simulink model "stepperMotorADRCFirstOrderDataCollection"  (R2026a)
settings: Solver=FixedStepDiscrete  StopTime=0.06  FixedStep=5e-9
undefined symbols (not defined in the file): ADC_Offset, adc_volts_per_count, alpha_iqd, alpha_s, beta_iqd, beta_s, biq, bs, convert_adc_to_integer, electricalRadiansPerCount, gam_iqd, gam_s, k1_iqd, k1_s, KPth, loadcell_decode_gain, mechanicalRadiansPerCount, precise_step_radians, PWMVoltage, theta_ref
libraries: simulink x2, mcbeeMathTransformLib x2, hdlsllib x1
settings Model: DataTypeOverride=Off  Creator=mike  LastModifiedBy=drew
settings OptimizationCC: ConditionallyExecuteInputs=off
settings DebuggingCC: ParameterPrecisionLossMsg=none
settings HardwareCC: ProdHWDeviceType=ASIC/FPGA->ASIC/FPGA  TargetBitPerLong=64.0  TargetBitPerPointer=64.0  TargetBitPerSizeT=64.0  TargetBitPerPtrDiffT=64.0  TargetLongLongMode=on  TargetIntDivRoundTo=Zero  TargetEndianess=LittleEndian  TargetWordSize=64.0  TargetHWDeviceType=Custom Processor->MATLAB Host Computer  ProdEqTarget=off

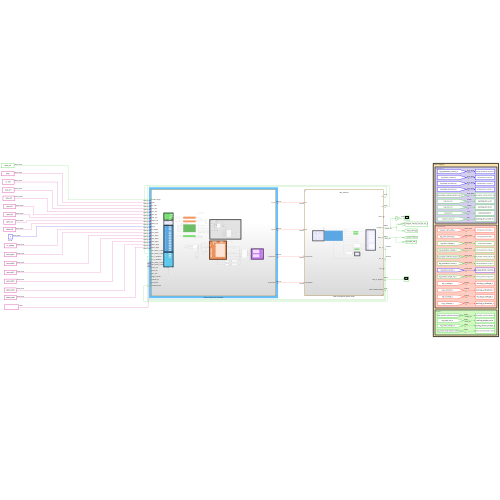
[thumbnail: Simulink's stored preview of the top-level diagram]
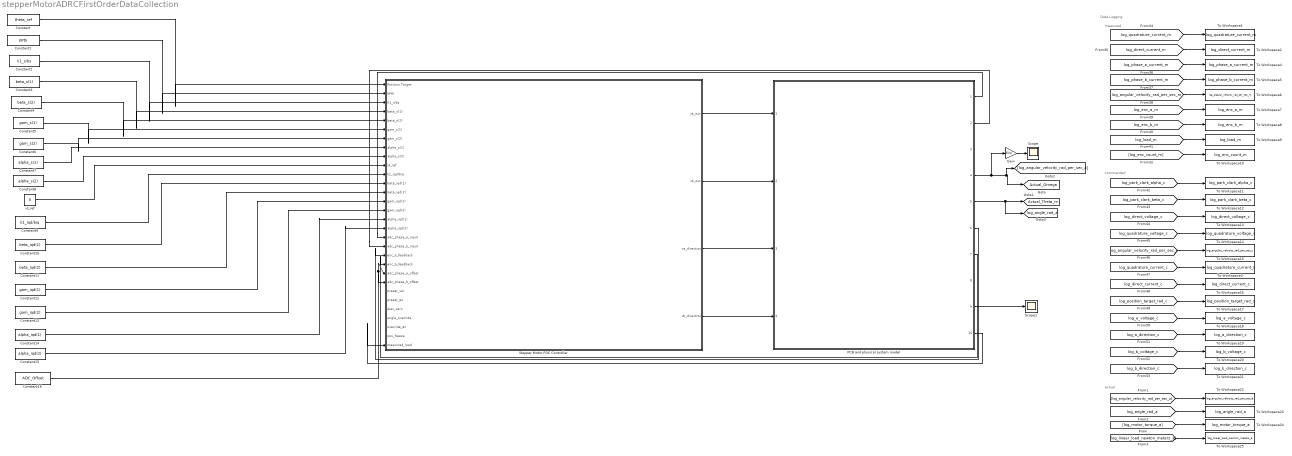
== system stepperMotorADRCFirstOrderDataCollection ==
  note: actual
  note: commanded
  note: measured
  note: Data Logging
  Constant : Constant  Value=theta_ref  OutDataTypeStr=PosType  SampleTime=-1
  Constant1 : Constant  Value=KPth  OutDataTypeStr=ParamType
  Constant10 : Constant  Value=beta_iqd(1)  OutDataTypeStr=ParamType
  Constant11 : Constant  Value=beta_iqd(2)  OutDataTypeStr=ParamType
  Constant12 : Constant  Value=gam_iqd(1)  OutDataTypeStr=ParamType
  Constant13 : Constant  Value=gam_iqd(2)  OutDataTypeStr=ParamType
  Constant14 : Constant  Value=alpha_iqd(1)  OutDataTypeStr=ParamType
  Constant15 : Constant  Value=alpha_iqd(2)  OutDataTypeStr=ParamType
  Constant16 : Constant  Value=ADC_Offset
  Constant2 : Constant  Value=k1_s/bs  OutDataTypeStr=ParamType
  Constant3 : Constant  Value=beta_s(1)  OutDataTypeStr=ParamType
  Constant4 : Constant  Value=beta_s(2)  OutDataTypeStr=ParamType
  Constant5 : Constant  Value=gam_s(1)  OutDataTypeStr=ParamType
  Constant6 : Constant  Value=gam_s(2)  OutDataTypeStr=ParamType
  Constant7 : Constant  Value=alpha_s(1)  OutDataTypeStr=ParamType
  Constant8 : Constant  Value=alpha_s(2)  OutDataTypeStr=ParamType
  Constant9 : Constant  Value=k1_iqd/biq  OutDataTypeStr=ParamType
  Gain : Gain  Gain=30/pi
  PCB and physical system model : Subsystem  ReferencedSubsystem=adrc_harness
  Scope : Scope
      settings: ActiveDisplayYMinimum=-42.844001916029548  ActiveDisplayYMaximum=385.596017244266  DataLoggingVariableName=ScopeData21
  Scope1 : Scope
      settings: Title=Actual Motor Position (Degrees)  ActiveDisplayYMinimum=117.68063353400193  ActiveDisplayYMaximum=118.08892845238269  YLabel=Degrees  DataLoggingVariableName=ScopeData8
  Stepper Motor FOC Controller : Subsystem
  To Workspace1 : ToWorkspace  VariableName=log_quadrature_current_m  SaveFormat=Timeseries  SampleTime=-1
  To Workspace10 : ToWorkspace  VariableName=log_enc_count_m  SaveFormat=Timeseries  SampleTime=-1
  To Workspace11 : ToWorkspace  VariableName=log_park_clark_alpha_c  SaveFormat=Timeseries  SampleTime=-1
  To Workspace12 : ToWorkspace  VariableName=log_park_clark_beta_c  SaveFormat=Timeseries  SampleTime=-1
  To Workspace13 : ToWorkspace  VariableName=log_direct_voltage_c  SaveFormat=Timeseries  SampleTime=-1
  To Workspace14 : ToWorkspace  VariableName=log_quadrature_voltage_c  SaveFormat=Timeseries  SampleTime=-1
  To Workspace15 : ToWorkspace  VariableName=log_angular_velocity_rad_per_sec_c  SaveFormat=Timeseries  SampleTime=-1
  To Workspace16 : ToWorkspace  VariableName=log_direct_current_c  SaveFormat=Timeseries  SampleTime=-1
  To Workspace17 : ToWorkspace  VariableName=log_position_target_rad_c  SaveFormat=Timeseries  SampleTime=-1
  To Workspace18 : ToWorkspace  VariableName=log_a_voltage_c  SaveFormat=Timeseries  SampleTime=-1
  To Workspace19 : ToWorkspace  VariableName=log_a_direction_c  SaveFormat=Timeseries  SampleTime=-1
  To Workspace2 : ToWorkspace  VariableName=log_direct_current_m  SaveFormat=Timeseries  SampleTime=-1
  To Workspace20 : ToWorkspace  VariableName=log_b_voltage_c  SaveFormat=Timeseries  SampleTime=-1
  To Workspace21 : ToWorkspace  VariableName=log_b_direction_c  SaveFormat=Timeseries  SampleTime=-1
  To Workspace22 : ToWorkspace  VariableName=log_angular_velocity_rad_per_sec_a  SaveFormat=Timeseries  SampleTime=-1
  To Workspace23 : ToWorkspace  VariableName=log_angle_rad_a  SaveFormat=Timeseries  SampleTime=-1
  To Workspace24 : ToWorkspace  VariableName=log_motor_torque_a  SaveFormat=Timeseries  SampleTime=-1
  To Workspace25 : ToWorkspace  VariableName=log_linear_load_newton_meters_a  SaveFormat=Timeseries  SampleTime=-1
  To Workspace3 : ToWorkspace  VariableName=log_quadrature_current_c  SaveFormat=Timeseries  SampleTime=-1
  To Workspace4 : ToWorkspace  VariableName=log_phase_a_current_m  SaveFormat=Timeseries  SampleTime=-1
  To Workspace5 : ToWorkspace  VariableName=log_phase_b_current_m  SaveFormat=Timeseries  SampleTime=-1
  To Workspace6 : ToWorkspace  VariableName=log_angular_velocity_rad_per_sec_m  SaveFormat=Timeseries  SampleTime=-1
  To Workspace7 : ToWorkspace  VariableName=log_enc_a_m  SaveFormat=Timeseries  SampleTime=-1
  To Workspace8 : ToWorkspace  VariableName=log_enc_b_m  SaveFormat=Timeseries  SampleTime=-1
  To Workspace9 : ToWorkspace  VariableName=log_load_m  SaveFormat=Timeseries  SampleTime=-1
  id_ref : Constant  Value=0  OutDataTypeStr=ParamType  SampleTime=-1
  tag scope: Actual_Omega=global, Actual_Theta_m=global, log_angle_rad_a=global
  wires:
  Constant/1 -> Stepper Motor FOC Controller/1(Position Target)
  Constant1/1 -> Stepper Motor FOC Controller/2(KPth)
  Constant2/1 -> Stepper Motor FOC Controller/3(K1_s/bs)
  Constant3/1 -> Stepper Motor FOC Controller/4(beta_s(1))
  Constant4/1 -> Stepper Motor FOC Controller/5(beta_s(2))
  Constant5/1 -> Stepper Motor FOC Controller/6(gam_s(1))
  Constant6/1 -> Stepper Motor FOC Controller/7(gam_s(2))
  Constant7/1 -> Stepper Motor FOC Controller/8(alpha_s(1))
  Constant8/1 -> Stepper Motor FOC Controller/9(alpha_s(2))
  id_ref/1 -> Stepper Motor FOC Controller/10(id_ref)
  Constant9/1 -> Stepper Motor FOC Controller/11(k1_iqd/biq)
  Constant10/1 -> Stepper Motor FOC Controller/12(beta_iqd(1))
  Constant11/1 -> Stepper Motor FOC Controller/13(beta_iqd(2))
  Constant12/1 -> Stepper Motor FOC Controller/14(gam_iqd(1))
  Constant13/1 -> Stepper Motor FOC Controller/15(gam_iqd(2))
  Constant14/1 -> Stepper Motor FOC Controller/16(alpha_iqd(1))
  Constant15/1 -> Stepper Motor FOC Controller/17(alpha_iqd(2))
  Stepper Motor FOC Controller/1(va_out) -> PCB and physical system model/1
  Stepper Motor FOC Controller/2(vb_out) -> PCB and physical system model/2
  PCB and physical system model/7 -> Stepper Motor FOC Controller/21(enc_b_feedback)
  PCB and physical system model/6 -> Stepper Motor FOC Controller/20(enc_a_feedback)
  PCB and physical system model/1 -> Stepper Motor FOC Controller/18(adc_phase_a_input)
  PCB and physical system model/2 -> Stepper Motor FOC Controller/19(adc_phase_b_input)
  PCB and physical system model/5 -> [log_angle_rad_a], [Actual_Theta_m]
  PCB and physical system model/9 -> Scope1/1
  Constant16/1 -> Stepper Motor FOC Controller/22(adc_phase_a_offset), Stepper Motor FOC Controller/23(adc_phase_b_offset)
  Stepper Motor FOC Controller/3(va_direction) -> PCB and physical system model/3
  Stepper Motor FOC Controller/4(vb_direction) -> PCB and physical system model/4
  PCB and physical system model/4 -> [log_angular_velocity_rad_per_sec_a], [Actual_Omega], Gain/1
  PCB and physical system model/10 -> Stepper Motor FOC Controller/30(measured_load)
  Gain/1 -> Scope/1
  [log_motor_torque_a] -> To Workspace24/1
  [log_direct_current_c] -> To Workspace16/1
  [log_a_direction_c] -> To Workspace19/1
  [log_quadrature_voltage_c] -> To Workspace14/1
  [log_park_clark_alpha_c] -> To Workspace11/1
  [log_quadrature_current_c] -> To Workspace3/1
  [log_b_direction_c] -> To Workspace21/1
  [log_a_voltage_c] -> To Workspace18/1
  [log_direct_voltage_c] -> To Workspace13/1
  [log_quadrature_current_m] -> To Workspace1/1
  [log_angular_velocity_rad_per_sec_c] -> To Workspace15/1
  [log_phase_a_current_m] -> To Workspace4/1
  [log_direct_current_m] -> To Workspace2/1
  [log_enc_count_m] -> To Workspace10/1
  [log_load_m] -> To Workspace9/1
  [log_enc_b_m] -> To Workspace8/1
  [log_position_target_rad_c] -> To Workspace17/1
  [log_enc_a_m] -> To Workspace7/1
  [log_park_clark_beta_c] -> To Workspace12/1
  [log_b_voltage_c] -> To Workspace20/1
  [log_phase_b_current_m] -> To Workspace5/1
  [log_angular_velocity_rad_per_sec_m] -> To Workspace6/1
  [log_angular_velocity_rad_per_sec_a] -> To Workspace22/1
  [log_angle_rad_a] -> To Workspace23/1
  [log_linear_load_newton_meters_a] -> To Workspace25/1

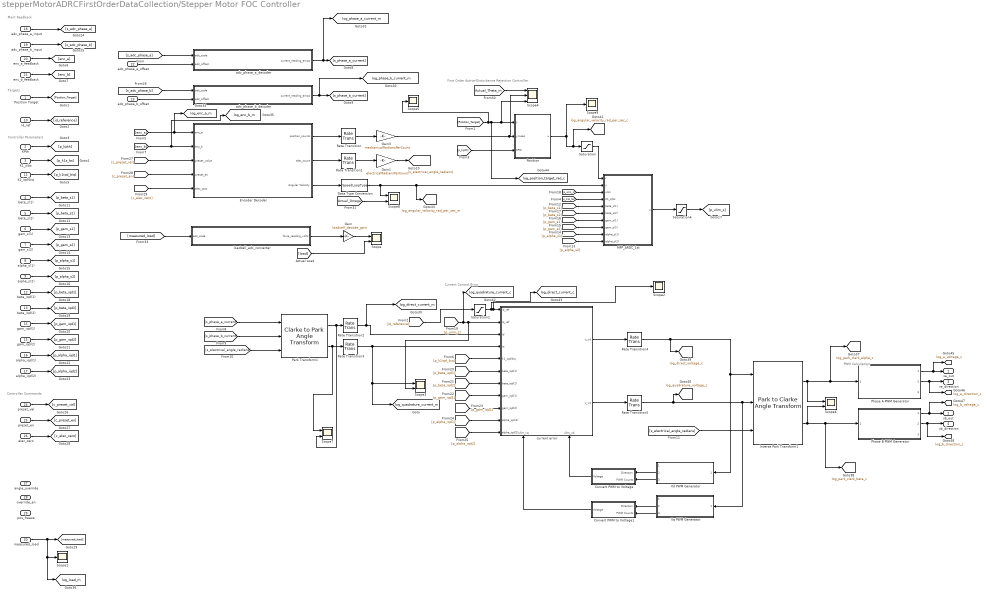
== system stepperMotorADRCFirstOrderDataCollection/Stepper Motor FOC Controller ==
  note: PWM Calculation
  note: Current Control Error
  note: Controller Commands
  note: Controller Parameters
  note: Targets
  note: Plant Feedback
  note: First Order Active-Disturbance Rejection Controller
  Position Target : Inport  OutDataTypeStr=PosType
  KPth : Inport  Port=2  OutDataTypeStr=ParamType
  K1_s/bs : Inport  Port=3  OutDataTypeStr=ParamType
  beta_s(1) : Inport  Port=4  OutDataTypeStr=ParamType
  beta_s(2) : Inport  Port=5  OutDataTypeStr=ParamType
  gam_s(1) : Inport  Port=6  OutDataTypeStr=ParamType
  gam_s(2) : Inport  Port=7  OutDataTypeStr=ParamType
  alpha_s(1) : Inport  Port=8  OutDataTypeStr=ParamType
  alpha_s(2) : Inport  Port=9  OutDataTypeStr=ParamType
  id_ref : Inport  Port=10  OutDataTypeStr=ParamType
  k1_iqd/biq : Inport  Port=11  OutDataTypeStr=ParamType
  beta_iqd(1) : Inport  Port=12  OutDataTypeStr=ParamType
  beta_iqd(2) : Inport  Port=13  OutDataTypeStr=ParamType
  gam_iqd(1) : Inport  Port=14  OutDataTypeStr=ParamType
  gam_iqd(2) : Inport  Port=15  OutDataTypeStr=ParamType
  alpha_iqd(1) : Inport  Port=16  OutDataTypeStr=ParamType
  alpha_iqd(2) : Inport  Port=17  OutDataTypeStr=ParamType
  adc_phase_a_input : Inport  Port=18
  adc_phase_b_input : Inport  Port=19
  enc_a_feedback : Inport  Port=20
  enc_b_feedback : Inport  Port=21
  adc_phase_a_offset : Inport  Port=22  OutDataTypeStr=uint16
  adc_phase_b_offset : Inport  Port=23  OutDataTypeStr=uint16
  preset_val : Inport  Port=24  OutDataTypeStr=fixdt(1,32,0)
  preset_en : Inport  Port=25  OutDataTypeStr=boolean
  elec_zero : Inport  Port=26  OutDataTypeStr=boolean
  angle_override : Inport  Port=27  OutDataTypeStr=uint16
  override_en : Inport  Port=28  OutDataTypeStr=boolean
  pos_freeze : Inport  Port=29  OutDataTypeStr=boolean
  measured_load : Inport  Port=30
  Convert PWM to Voltage : Subsystem
  Convert PWM to Voltage1 : Subsystem
  Data Type Conversion : DataTypeConversion  OutDataTypeStr=SpeedLoopType  SaturateOnIntegerOverflow=off  RndMeth=Floor
  Encoder Decoder : Subsystem
  Gain : Gain  Gain=loadcell_decode_gain  OutDataTypeStr=ParamType
  Gain1 : Gain  Gain=electricalRadiansPerCount  OutDataTypeStr=PosType  SaturateOnIntegerOverflow=on
  Gain3 : Gain  Gain=mechanicalRadiansPerCount  OutDataTypeStr=PosType  SaturateOnIntegerOverflow=on
  Inverse Park Transform1 : mcbeeMathTransformLib/Park to Clarke Angle Transform  AxisAlignment=D-axis  UseWithEmbedded=on  PhaseInput=Two inputs  ThetaInput=Electrical position  AngleInput=Radians  N_points=1024
      settings: LibrarySourceBlock=mcbhdllib/Controls/Math Transforms/Inverse Park Transform
  MFP_ARDC_1st : Subsystem
  Park Transform1 : mcbeeMathTransformLib/Clarke to Park Angle Transform  AxisAlignment=D-axis  UseWithEmbedded=on  PhaseInput=Two inputs  ThetaInput=Electrical position  AngleInput=Radians  N_points=1024
      settings: LibrarySourceBlock=mcbhdllib/Controls/Math Transforms/Park Transform
  Phase A PWM Generator : Subsystem  ReferencedSubsystem=PWM_Generator
  Phase B PWM Generator : Subsystem  ReferencedSubsystem=PWM_Generator
  "Position " : Subsystem
  Rate Transition{,1..3} (4 alike) : RateTransition  OutPortSampleTime=2e-5
  Rate Transition4 : RateTransition  OutPortSampleTime=1e-7
  Rate Transition5 : RateTransition  OutPortSampleTime=1e-7
  Saturation : Saturate  UpperLimit=35.5  LowerLimit=-35.5
  Saturation2 : Saturate  UpperLimit=2.4  LowerLimit=-2.4  OutDataTypeStr=ParamType
  Saturation4 : Saturate  UpperLimit=4.16  LowerLimit=-4.16
  Scope{,3,6..8} (5 alike) : Scope  NumInputPorts=2
      Scope settings: Title=Calculated Load and Torque Load  ActiveDisplayYMinimum=-0.011365323760298198  ActiveDisplayYMaximum=0.10228791384268379
      Scope3 settings: Title=Measured Iq vs Iq Reference  ActiveDisplayYMinimum=-7.8918533325195312  ActiveDisplayYMaximum=11.987983703613281  YLabel=Amps  DataLoggingVariableName=ScopeData20
      Scope6 settings: Title="Output  Voltages"  ActiveDisplayYMinimum=-1  ActiveDisplayYMaximum=1  DataLoggingVariableName=ScopeData9  DataLoggingSaveFormat=Array
      Scope7 settings: ActiveDisplayYMinimum=-1  ActiveDisplayYMaximum=1  DataLoggingVariableName=ScopeData26
      Scope8 settings: Title=Calculated and Actual Velocity  ActiveDisplayYMinimum=5.2986835943204227  ActiveDisplayYMaximum=29.84236950740636  YLabel=Radians/Second  DataLoggingVariableName=ScopeData23  DataLoggingSaveFormat=Array
  Scope{1..2,5,9} (4 alike) : Scope
      Scope1 settings: ActiveDisplayYMinimum=-1  ActiveDisplayYMaximum=1  DataLoggingVariableName=ScopeData5
      Scope2 settings: ActiveDisplayYMinimum=-1  ActiveDisplayYMaximum=1  DataLoggingVariableName=ScopeData22
      Scope5 settings: ActiveDisplayYMinimum=-1  ActiveDisplayYMaximum=1  DataLoggingVariableName=ScopeData25
      Scope9 settings: Title=Output of Position Controller  ActiveDisplayYMinimum=21899.960541585759  ActiveDisplayYMaximum=43949.960541585751  YLabel=Radians  DataLoggingVariableName=ScopeData24  DataLoggingSaveFormat=Array
  Scope4 : Scope  NumInputPorts=3
      settings: Title=Position Debugging  ActiveDisplayYMinimum=-0.035609373496401926  ActiveDisplayYMaximum=0.32048436146761738  YLabel=Radians  DataLoggingVariableName=ScopeData7  DataLoggingSaveFormat=Array
  Vd PWM Generator : Subsystem  ReferencedSubsystem=PWM_Generator
  Vq PWM Generator : Subsystem  ReferencedSubsystem=PWM_Generator
  adc_phase_a_decoder : Subsystem
  adc_phase_b_decoder : Subsystem
  current error : Subsystem
      settings: PortSchema="{\"entries\":[{\"content\":{\"sides\":[{\"content\":{\"connectorIds\":[\"In1\",\"In2\",\"In3\",\"In4\",\"In5\",\"In6\",\"In7\",\"In8\",\"In9\",\"In10\",\"In11\"]},\"type\":\"ConnectorPlacement.EquallySpacedRectSide\",\"uuid\":\"1b67f1ba-d970-4a72-948b-8a645885f311\"},{\"content\":{\"connectorIds\":[\"Out1\",\"Out2\"],\"side\":\"RIGHT\"},\"type\":\"ConnectorPlacement.EquallySpacedRectSide\",\"uuid\":\"43bd9de9-c038-41d9-a38f-2b3bf68f84b7\"},{\"content\":{\"side\":\"TOP\"},\"type\":\"ConnectorPlacement.EquallySpacedRectSide\",\"uuid\":\"199b5c60-7e13-4435-9b33-d3faaa781c81\"},{\"content\":{\"connectorIds\":[\"In12\",\"In13\"],\"side\":\"BOTTOM\"},\"type\":\"ConnectorPlacement.EquallySpacedRectSide\",\"uuid\":\"8463aca4-e427-4dc0-a0b4-e373bcd68b49\"}]},\"type\":\"ConnectorPlacement.EquallySpacedConnector\",\"uuid\":\"7665834e-14df-482a-91d4-36c3c32286ac\"}],\"packageUris\":[\"http://schema.mathworks.com/mf0/Connector/R2020b\"],\"version\":\"1.0\"}"
  loadcell_adc_converter : Subsystem
  va_out : Outport  OutDataTypeStr=boolean
  vb_out : Outport  Port=2  OutDataTypeStr=boolean
  va_direction : Outport  Port=3  OutDataTypeStr=boolean
  vb_direction : Outport  Port=4  OutDataTypeStr=boolean
  tag scope: log_a_direction_c=global, log_a_voltage_c=global, log_angular_velocity_rad_per_sec_c=global, log_angular_velocity_rad_per_sec_m=global, log_b_direction_c=global, log_b_voltage_c=global, log_direct_current_c=global, log_direct_current_m=global, log_direct_voltage_c=global, log_enc_a_m=global, log_enc_b_m=global, log_load_m=global, log_park_clark_alpha_c=global, log_park_clark_beta_c=global, log_phase_a_current_m=global, log_phase_b_current_m=global, log_position_target_rad_c=global, log_quadrature_current_c=global, log_quadrature_current_m=global, log_quadrature_voltage_c=global
  wires:
  [Position_Target] -> Scope5/1, [log_position_target_rad_c], Scope4/3, "Position "/1(y)
  Inverse Park Transform1/1 -> [log_park_clark_alpha_c], Phase A PWM Generator/1, Scope6/1
  Position Target/1 -> [Position_Target]
  id_ref/1 -> [id_reference]
  [p_kpth] -> "Position "/3(KPth)
  KPth/1 -> [p_kpth]
  [p_k1s_bs] -> MFP_ARDC_1st/4(K1_s/bs)
  K1_s/bs/1 -> [p_k1s_bs]
  [p_k1iqd_biq] -> current error/5(k1_iqd/biq)
  k1_iqd/biq/1 -> [p_k1iqd_biq]
  adc_phase_a_offset/1 -> adc_phase_a_decoder/2(adc_offset)
  adc_phase_b_offset/1 -> adc_phase_b_decoder/2(adc_offset)
  enc_a_feedback/1 -> [enc_a]
  enc_b_feedback/1 -> [enc_b]
  [enc_a] -> [log_enc_a_m], Encoder Decoder/1(enc_a)
  [enc_b] -> [log_enc_b_m], Encoder Decoder/2(enc_b)
  adc_phase_a_decoder/1(current_reading_amps) -> [log_phase_a_current_m], [s_phase_a_current]
  adc_phase_b_decoder/1(current_reading_amps) -> [log_phase_b_current_m], [s_phase_b_current]
  [s_phase_a_current] -> Park Transform1/1
  [s_phase_b_current] -> Park Transform1/2
  [s_electrical_angle_radians] -> Park Transform1/3
  [s_electrical_angle_radians] -> Inverse Park Transform1/3
  [p_beta_s1] -> MFP_ARDC_1st/5(beta_s(1))
  [p_beta_s2] -> MFP_ARDC_1st/6(beta_s(2))
  [p_gam_s1] -> MFP_ARDC_1st/7(gam_s(1))
  [p_gam_s2] -> MFP_ARDC_1st/8(gam_s(2))
  [p_alpha_s1] -> MFP_ARDC_1st/9(alpha_s(1))
  [p_alpha_s2] -> MFP_ARDC_1st/10(alpha_s(2))
  alpha_s(2)/1 -> [p_alpha_s2]
  alpha_s(1)/1 -> [p_alpha_s1]
  gam_s(2)/1 -> [p_gam_s2]
  gam_s(1)/1 -> [p_gam_s1]
  beta_s(2)/1 -> [p_beta_s2]
  beta_s(1)/1 -> [p_beta_s1]
  MFP_ARDC_1st/1(u) -> Saturation4/1
  [p_ulim_s] -> MFP_ARDC_1st/3(ulim)
  beta_iqd(1)/1 -> [p_beta_iqd1]
  beta_iqd(2)/1 -> [p_beta_iqd2]
  [p_beta_iqd2] -> current error/7(beta_iqd(2))
  [p_beta_iqd1] -> current error/6(beta_iqd(1))
  gam_iqd(2)/1 -> [p_gam_iqd2]
  gam_iqd(1)/1 -> [p_gam_iqd1]
  [p_gam_iqd1] -> current error/8(gam_iqd(1))
  [p_gam_iqd2] -> current error/9(gam_iqd(2))
  [p_alpha_iqd1] -> current error/10(alpha_iqd(1))
  [p_alpha_iqd2] -> current error/11(alpha_iqd(2))
  alpha_iqd(1)/1 -> [p_alpha_iqd1]
  alpha_iqd(2)/1 -> [p_alpha_iqd2]
  adc_phase_a_input/1 -> [s_adc_phase_a]
  adc_phase_b_input/1 -> [s_adc_phase_b]
  [s_adc_phase_a] -> adc_phase_a_decoder/1(adc_code)
  [s_adc_phase_b] -> adc_phase_b_decoder/1(adc_code)
  [c_elec_zero] -> Encoder Decoder/5(elec_zero)
  [c_preset_en] -> Encoder Decoder/4(preset_en)
  [c_preset_val] -> Encoder Decoder/3(preset_value)
  elec_zero/1 -> [c_elec_zero]
  preset_en/1 -> [c_preset_en]
  preset_val/1 -> [c_preset_val]
  Saturation2/1 -> Scope2/1, [log_direct_current_c], current error/1(id_ref)
  Rate Transition/1 -> Gain3/1
  Rate Transition1/1 -> Gain1/1
  Gain1/1 -> [s_electrical_angle_radians]
  Gain3/1 -> "Position "/2(ymeas), Scope4/2
  current error/1(u_vd) -> Rate Transition4/1
  Saturation4/1 -> [p_ulim_s]
  Park Transform1/1 -> Scope7/2, Rate Transition2/1
  Park Transform1/2 -> Scope7/1, Rate Transition3/1
  current error/2(u_vq) -> Rate Transition5/1
  Encoder Decoder/1(position_counts) -> Rate Transition/1
  Encoder Decoder/2(elec_count) -> Rate Transition1/1
  "Position "/1(u) -> [log_angular_velocity_rad_per_sec_c], Saturation/1, Scope9/1
  Encoder Decoder/3(Angular Velocity) -> Data Type Conversion/1
  Phase A PWM Generator/1 -> [log_a_voltage_c], va_out/1
  Phase A PWM Generator/2 -> [log_a_direction_c], va_direction/1
  Phase B PWM Generator/2 -> [log_b_direction_c], vb_direction/1
  Phase B PWM Generator/1 -> [log_b_voltage_c], vb_out/1
  Convert PWM to Voltage1/1(Voltage) -> current error/12(ulim_vq)
  Rate Transition4/1 -> [log_direct_voltage_c], Vd PWM Generator/1, Inverse Park Transform1/1
  Rate Transition5/1 -> [log_quadrature_voltage_c], Inverse Park Transform1/2, Vq PWM Generator/1
  [p_ulim_s] -> [log_quadrature_current_c], Scope3/2, current error/2(iq_ref)
  Data Type Conversion/1 -> [log_angular_velocity_rad_per_sec_m], MFP_ARDC_1st/2(y), Scope8/1
  Inverse Park Transform1/2 -> Scope6/2, [log_park_clark_beta_c], Phase B PWM Generator/1
  [Actual_Theta_m] -> Scope4/1
  Convert PWM to Voltage/1(Voltage) -> current error/13(ulim_vd)
  Vd PWM Generator/2 -> Convert PWM to Voltage/1(Direction)
  Vd PWM Generator/3 -> Convert PWM to Voltage/2(PWM Counts)
  Vq PWM Generator/3 -> Convert PWM to Voltage1/2(PWM Counts)
  Vq PWM Generator/2 -> Convert PWM to Voltage1/1(Direction)
  measured_load/1 -> [log_load_m], Scope1/1, [measured_load]
  loadcell_adc_converter/1(force_reading_volts) -> Gain/1
  [load] -> Scope/2
  [measured_load] -> loadcell_adc_converter/1(adc_code)
  Saturation/1 -> MFP_ARDC_1st/1(r)
  [Actual_Omega] -> Scope8/2
  Rate Transition3/1 -> [log_quadrature_current_m], Scope3/1, current error/4(iq)
  Rate Transition2/1 -> [log_direct_current_m], current error/3(id)
  [id_reference] -> Saturation2/1
  Gain/1 -> Scope/1

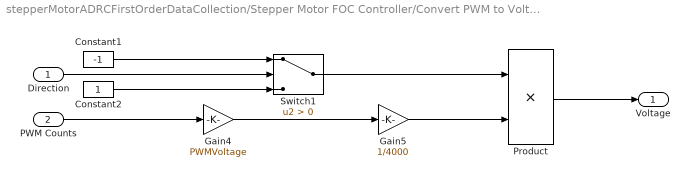
== system stepperMotorADRCFirstOrderDataCollection/Stepper Motor FOC Controller/Convert PWM to Voltage ==
  Direction : Inport
  PWM Counts : Inport  Port=2
  Constant1 : Constant  Value=-1
  Constant2 : Constant
  Gain4 : Gain  Gain=PWMVoltage
  Gain5 : Gain  Gain=1/4000
  Product : Product
  Switch1 : Switch  Criteria=u2 > Threshold  SaturateOnIntegerOverflow=off  InputSameDT=off
  Voltage : Outport
  wires:
  Gain4/1 -> Gain5/1
  Gain5/1 -> Product/2
  Switch1/1 -> Product/1
  Constant1/1 -> Switch1/1
  Constant2/1 -> Switch1/3
  PWM Counts/1 -> Gain4/1
  Direction/1 -> Switch1/2
  Product/1 -> Voltage/1

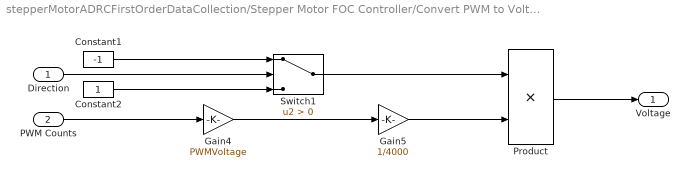
== system stepperMotorADRCFirstOrderDataCollection/Stepper Motor FOC Controller/Convert PWM to Voltage1 ==
  Direction : Inport
  PWM Counts : Inport  Port=2
  Constant1 : Constant  Value=-1
  Constant2 : Constant
  Gain4 : Gain  Gain=PWMVoltage
  Gain5 : Gain  Gain=1/4000
  Product : Product
  Switch1 : Switch  Criteria=u2 > Threshold  SaturateOnIntegerOverflow=off  InputSameDT=off
  Voltage : Outport
  wires:
  Gain4/1 -> Gain5/1
  Gain5/1 -> Product/2
  Switch1/1 -> Product/1
  Constant1/1 -> Switch1/1
  Constant2/1 -> Switch1/3
  PWM Counts/1 -> Gain4/1
  Direction/1 -> Switch1/2
  Product/1 -> Voltage/1

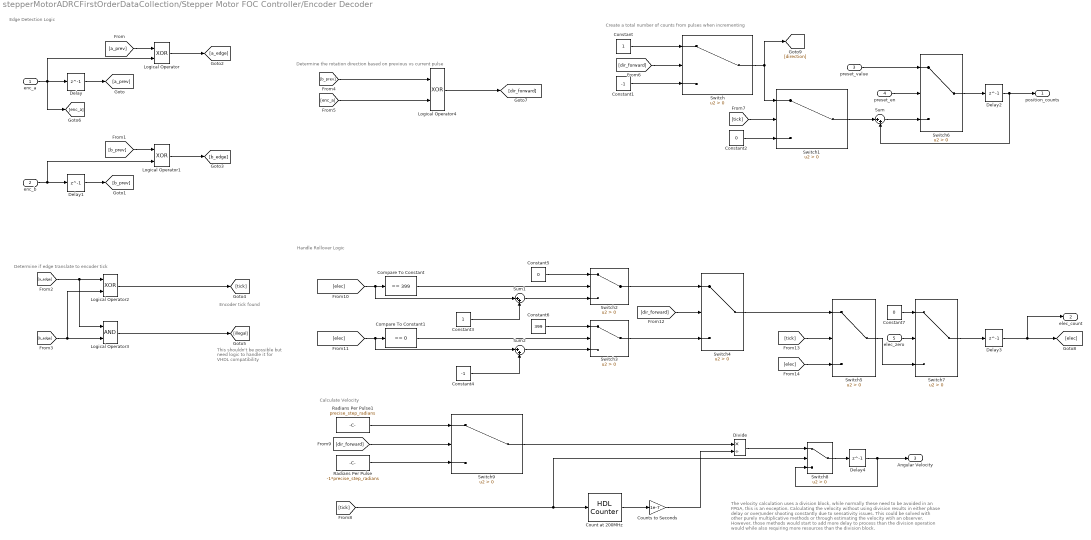
== system stepperMotorADRCFirstOrderDataCollection/Stepper Motor FOC Controller/Encoder Decoder ==
  note: The velocity calculation uses a division block, while normally these need to be avoided in an FPGA, this is an exception. Calculating the velocity without using division results in either phase delay or over/under shooting constantly due to sensativity issues. This could be solved with other purely multiplicative methods or through estimating the velocity wtih an observer. However, those methods would start to add more delay to process than the division operation would while also requiring more resources than the division block.
  note: Calculate Velocity
  note: Handle Rollover Logic
  note: Create a total number of counts from pulses when incrementing
  note: Determine the rotation direction based on previous vs current pulse
  note: Encoder tick found
  note: Determine if edge translate to encoder tick
  note: Edge Detection Logic
  note: This shouldn't be possible but need logic to handle it for VHDL compatibility
  enc_a : Inport  OutDataTypeStr=boolean
  enc_b : Inport  Port=2  OutDataTypeStr=boolean
  preset_value : Inport  Port=3  OutDataTypeStr=fixdt(1,32,0)
  preset_en : Inport  Port=4  OutDataTypeStr=boolean
  elec_zero : Inport  Port=5  OutDataTypeStr=boolean
  Compare To Constant : simulink/Logic and Bit Operations/Compare To Constant  relop===  const=399  OutDataTypeStr=boolean
  Compare To Constant1 : simulink/Logic and Bit Operations/Compare To Constant  relop===  const=0  OutDataTypeStr=boolean
  Constant : Constant  OutDataTypeStr=int32
  Constant1 : Constant  Value=-1  OutDataTypeStr=int32
  Constant2 : Constant  Value=0  OutDataTypeStr=int32
  Constant3 : Constant  OutDataTypeStr=int32
  Constant4 : Constant  Value=-1  OutDataTypeStr=int32
  Constant5 : Constant  Value=0  OutDataTypeStr=int32
  Constant6 : Constant  Value=399  OutDataTypeStr=int32
  Constant7 : Constant  Value=0  OutDataTypeStr=int32
  Count at 200MHz : hdlsllib/Sources/HDL Counter  CountType=Count limited  CountInit=0  CountStep=1  CountMax=199999999  CountFromType=Initial value  CountFrom=0  CountResetPort=on  CountLoadPort=off  CountEnbPort=off  CountDirPort=off  CountHitOutputPort=off  CountDataType=Unsigned  CountWordLen=32  CountFracLen=0  CountSampTime=5e-9
  Counts to Seconds : Gain  Gain=1e-7  OutDataTypeStr=VelType
  Delay{,1..4} (5 alike) : Delay  DelayLength=1  InputProcessing=Columns as channels (frame based)  SampleTime=1e-7
  Divide : Product  Inputs=*/  OutDataTypeStr=VelType  SaturateOnIntegerOverflow=on
  Logical Operator{,1..2,4} (4 alike) : Logic  Operator=XOR  AllPortsSameDT=off  OutDataTypeStr=boolean
  Logical Operator3 : Logic  AllPortsSameDT=off  OutDataTypeStr=boolean
  Radians Per Pulse : Constant  Value=-1*precise_step_radians  OutDataTypeStr=VelType
  Radians Per Pulse1 : Constant  Value=precise_step_radians  OutDataTypeStr=VelType
  Sum : Sum  Inputs=|++  OutDataTypeStr=int32  SaturateOnIntegerOverflow=on
  Sum1 : Sum  Inputs=|++  OutDataTypeStr=int32
  Sum2 : Sum  Inputs=|++  OutDataTypeStr=int32
  Switch{,1..5} (6 alike) : Switch  Criteria=u2 > Threshold  SaturateOnIntegerOverflow=off  InputSameDT=off
  Switch6 : Switch  Criteria=u2 > Threshold  OutDataTypeStr=CountType  SaturateOnIntegerOverflow=off  InputSameDT=off
  Switch7 : Switch  Criteria=u2 > Threshold  OutDataTypeStr=CountType  SaturateOnIntegerOverflow=off  InputSameDT=off
  Switch8 : Switch  Criteria=u2 > Threshold  OutDataTypeStr=VelType  SaturateOnIntegerOverflow=off  InputSameDT=off
  Switch9 : Switch  Criteria=u2 > Threshold  OutDataTypeStr=VelType  SaturateOnIntegerOverflow=off  InputSameDT=off
  position_counts : Outport  OutDataTypeStr=CountType
  elec_count : Outport  Port=2  OutDataTypeStr=CountType
  Angular Velocity : Outport  Port=3  OutDataTypeStr=VelType
  wires:
  enc_b/1 -> Logical Operator1/2, Delay1/1
  enc_a/1 -> [enc_a], Logical Operator/2, Delay/1
  Delay/1 -> [a_prev]
  Delay1/1 -> [b_prev]
  [b_prev] -> Logical Operator1/1
  [a_prev] -> Logical Operator/1
  Logical Operator/1 -> [a_edge]
  Logical Operator1/1 -> [b_edge]
  [b_edge] -> Logical Operator3/2, Logical Operator2/2
  [a_edge] -> Logical Operator2/1, Logical Operator3/1
  Logical Operator2/1 -> [tick]
  Logical Operator3/1 -> [illegal]
  [b_prev] -> Logical Operator4/1
  [enc_a] -> Logical Operator4/2
  Logical Operator4/1 -> [dir_forward]
  Constant/1 -> Switch/1
  Constant1/1 -> Switch/3
  [dir_forward] -> Switch/2
  [tick] -> Switch1/2
  Constant2/1 -> Switch1/3
  Switch/1 -> Switch1/1, [direction]
  Switch1/1 -> Sum/1
  Delay2/1 -> position_counts/1, Sum/2
  Constant5/1 -> Switch2/1
  Compare To Constant1/1 -> Switch3/2
  Sum2/1 -> Switch3/3
  Sum1/1 -> Switch2/3
  Constant6/1 -> Switch3/1
  [elec] -> Sum2/1, Compare To Constant1/1
  [elec] -> Sum1/1, Compare To Constant/1
  Switch2/1 -> Switch4/1
  Constant3/1 -> Sum1/2
  Compare To Constant/1 -> Switch2/2
  Constant4/1 -> Sum2/2
  [dir_forward] -> Switch4/2
  Switch3/1 -> Switch4/3
  Switch4/1 -> Switch5/1
  [tick] -> Switch5/2
  [elec] -> Switch5/3
  Delay3/1 -> elec_count/1, [elec]
  Sum/1 -> Switch6/3
  Switch6/1 -> Delay2/1
  preset_en/1 -> Switch6/2
  preset_value/1 -> Switch6/1
  Constant7/1 -> Switch7/1
  elec_zero/1 -> Switch7/2
  Switch5/1 -> Switch7/3
  Switch7/1 -> Delay3/1
  Count at 200MHz/1 -> Counts to Seconds/1
  Switch8/1 -> Delay4/1
  Delay4/1 -> Angular Velocity/1, Switch8/3
  Counts to Seconds/1 -> Divide/2
  Switch9/1 -> Divide/1
  Radians Per Pulse/1 -> Switch9/3
  Radians Per Pulse1/1 -> Switch9/1
  Divide/1 -> Switch8/1
  [dir_forward] -> Switch9/2
  [tick] -> Switch8/2, Count at 200MHz/1

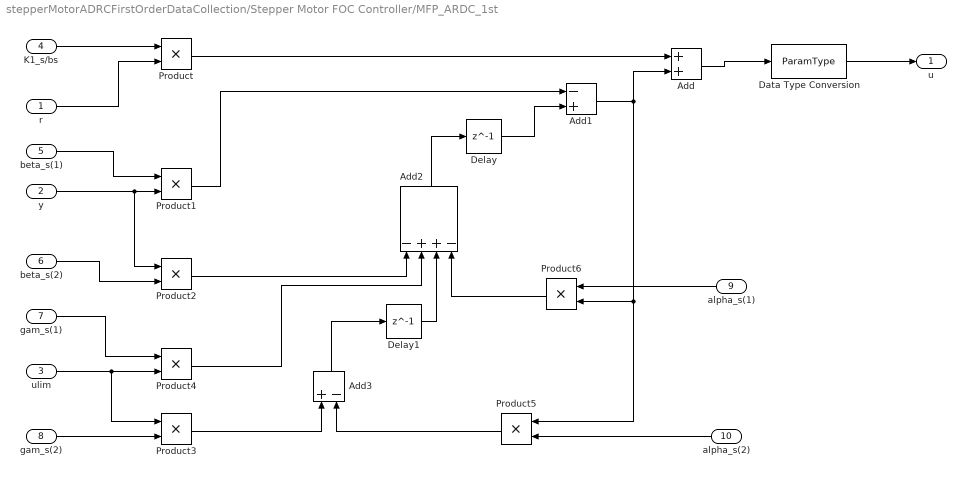
== system stepperMotorADRCFirstOrderDataCollection/Stepper Motor FOC Controller/MFP_ARDC_1st ==
  r : Inport  OutDataTypeStr=PosType
  y : Inport  Port=2  OutDataTypeStr=PosType
  ulim : Inport  Port=3  OutDataTypeStr=ParamType
  K1_s/bs : Inport  Port=4  OutDataTypeStr=ParamType
  beta_s(1) : Inport  Port=5  OutDataTypeStr=ParamType
  beta_s(2) : Inport  Port=6  OutDataTypeStr=ParamType
  gam_s(1) : Inport  Port=7  OutDataTypeStr=ParamType
  gam_s(2) : Inport  Port=8  OutDataTypeStr=ParamType
  alpha_s(1) : Inport  Port=9  OutDataTypeStr=ParamType
  alpha_s(2) : Inport  Port=10  OutDataTypeStr=ParamType
  Add : Sum  OutDataTypeStr=SpeedLoopType  SaturateOnIntegerOverflow=on
  Add1 : Sum  Inputs=-+  OutDataTypeStr=SpeedLoopType  SaturateOnIntegerOverflow=on
  Add2 : Sum  Inputs=-++-  OutDataTypeStr=SpeedLoopType  SaturateOnIntegerOverflow=on
  Add3 : Sum  Inputs=+-  OutDataTypeStr=SpeedLoopType  SaturateOnIntegerOverflow=on
  Data Type Conversion : DataTypeConversion  OutDataTypeStr=ParamType  RndMeth=Floor
  Delay : Delay  DelayLength=1  InitialCondition=0  SampleTime=2e-5
  Delay1 : Delay  DelayLength=1  InitialCondition=0  SampleTime=2e-5
  Product{,1..6} (7 alike) : Product  OutDataTypeStr=SpeedLoopType  SaturateOnIntegerOverflow=on
  u : Outport  OutDataTypeStr=ParamType
  wires:
  Add/1 -> Data Type Conversion/1
  Add3/1 -> Delay1/1
  Product4/1 -> Add2/2
  Product6/1 -> Add2/4
  Add1/1 -> Product5/1, Product6/2, Add/2
  Add2/1 -> Delay/1
  r/1 -> Product/2
  Delay1/1 -> Add2/3
  Product3/1 -> Add3/1
  ulim/1 -> Product3/1, Product4/2
  Product2/1 -> Add2/1
  Product5/1 -> Add3/2
  Delay/1 -> Add1/2
  Product1/1 -> Add1/1
  y/1 -> Product2/1, Product1/2
  K1_s/bs/1 -> Product/1
  Product/1 -> Add/1
  beta_s(1)/1 -> Product1/1
  beta_s(2)/1 -> Product2/2
  gam_s(1)/1 -> Product4/1
  gam_s(2)/1 -> Product3/2
  alpha_s(2)/1 -> Product5/2
  alpha_s(1)/1 -> Product6/1
  Data Type Conversion/1 -> u/1

== system stepperMotorADRCFirstOrderDataCollection/Stepper Motor FOC Controller/Position  ==
  y : Inport  OutDataTypeStr=PosType
  ymeas : Inport  Port=2  OutDataTypeStr=PosType
  KPth : Inport  Port=3  OutDataTypeStr=ParamType
  Product : Product  OutDataTypeStr=PosType  SaturateOnIntegerOverflow=on
  Sum : Sum  Inputs=|+-  OutDataTypeStr=PosType  SaturateOnIntegerOverflow=on
  u : Outport  OutDataTypeStr=PosType
  wires:
  y/1 -> Sum/1
  ymeas/1 -> Sum/2
  Sum/1 -> Product/2
  Product/1 -> u/1
  KPth/1 -> Product/1

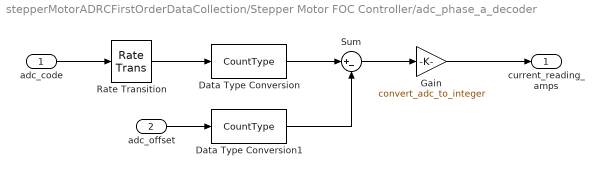
== system stepperMotorADRCFirstOrderDataCollection/Stepper Motor FOC Controller/adc_phase_a_decoder ==
  adc_code : Inport  OutMin=[0]  OutDataTypeStr=uint16
  adc_offset : Inport  Port=2  OutDataTypeStr=uint16
  Data Type Conversion : DataTypeConversion  OutDataTypeStr=CountType  RndMeth=Floor
  Data Type Conversion1 : DataTypeConversion  OutDataTypeStr=CountType  RndMeth=Floor
  Gain : Gain  Gain=convert_adc_to_integer  ParamDataTypeStr=fixdt(0,32,38)  OutDataTypeStr=ParamType  RndMeth=Nearest  SaturateOnIntegerOverflow=on
  Rate Transition : RateTransition  OutPortSampleTime=2e-5
  Sum : Sum  Inputs=|+-  OutDataTypeStr=CountType  AccumDataTypeStr=CountType  SaturateOnIntegerOverflow=on
  current_reading_amps : Outport  OutDataTypeStr=ParamType
  wires:
  adc_offset/1 -> Data Type Conversion1/1
  Data Type Conversion1/1 -> Sum/2
  Data Type Conversion/1 -> Sum/1
  Sum/1 -> Gain/1
  Gain/1 -> current_reading_amps/1
  adc_code/1 -> Rate Transition/1
  Rate Transition/1 -> Data Type Conversion/1

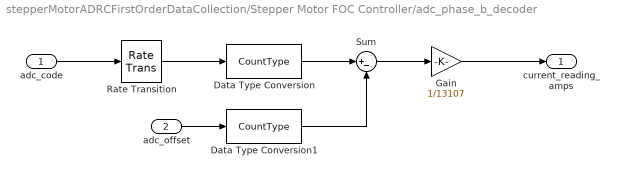
== system stepperMotorADRCFirstOrderDataCollection/Stepper Motor FOC Controller/adc_phase_b_decoder ==
  adc_code : Inport  OutMin=[0]  OutDataTypeStr=uint16
  adc_offset : Inport  Port=2  OutDataTypeStr=uint16
  Data Type Conversion : DataTypeConversion  OutDataTypeStr=CountType  RndMeth=Floor
  Data Type Conversion1 : DataTypeConversion  OutDataTypeStr=CountType  RndMeth=Floor
  Gain : Gain  Gain=1/13107  ParamDataTypeStr=fixdt(0,32,38)  OutDataTypeStr=ParamType  RndMeth=Nearest  SaturateOnIntegerOverflow=on
  Rate Transition : RateTransition  OutPortSampleTime=2e-5
  Sum : Sum  Inputs=|+-  OutDataTypeStr=CountType  AccumDataTypeStr=CountType  SaturateOnIntegerOverflow=on
  current_reading_amps : Outport  OutDataTypeStr=ParamType
  wires:
  adc_offset/1 -> Data Type Conversion1/1
  Data Type Conversion1/1 -> Sum/2
  Data Type Conversion/1 -> Sum/1
  Sum/1 -> Gain/1
  Gain/1 -> current_reading_amps/1
  Rate Transition/1 -> Data Type Conversion/1
  adc_code/1 -> Rate Transition/1

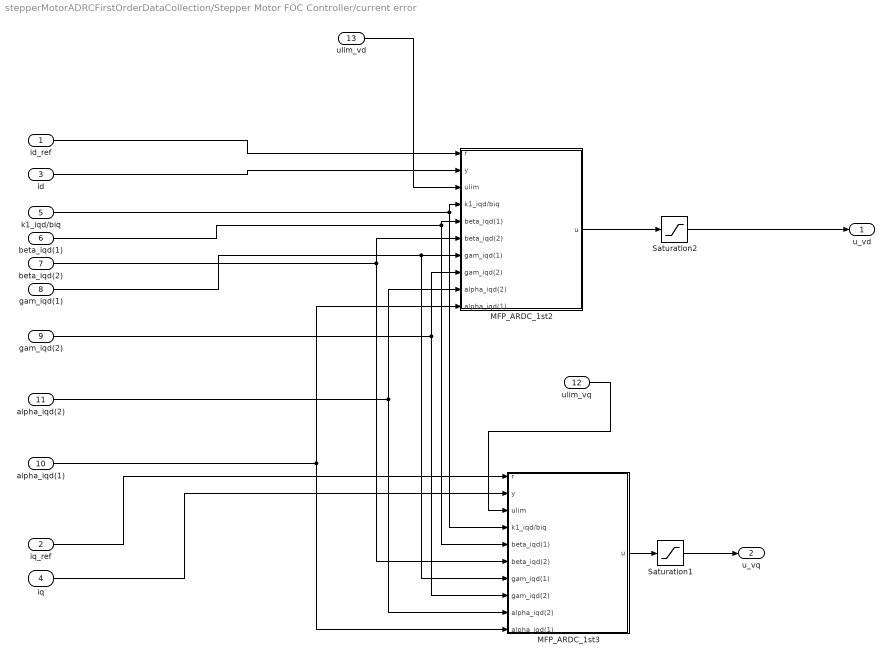
== system stepperMotorADRCFirstOrderDataCollection/Stepper Motor FOC Controller/current error ==
  id_ref : Inport  OutDataTypeStr=ParamType
  iq_ref : Inport  Port=2  OutDataTypeStr=ParamType
  id : Inport  Port=3  OutDataTypeStr=ParamType
  iq : Inport  Port=4  OutDataTypeStr=ParamType
  k1_iqd/biq : Inport  Port=5  OutDataTypeStr=ParamType
  beta_iqd(1) : Inport  Port=6  OutDataTypeStr=ParamType
  beta_iqd(2) : Inport  Port=7  OutDataTypeStr=ParamType
  gam_iqd(1) : Inport  Port=8  OutDataTypeStr=ParamType
  gam_iqd(2) : Inport  Port=9  OutDataTypeStr=ParamType
  alpha_iqd(1) : Inport  Port=10  OutDataTypeStr=ParamType
  alpha_iqd(2) : Inport  Port=11  OutDataTypeStr=ParamType
  ulim_vq : Inport  Port=12
  ulim_vd : Inport  Port=13
  MFP_ARDC_1st2 : Subsystem
  MFP_ARDC_1st3 : Subsystem
  Saturation1 : Saturate  UpperLimit=PWMVoltage  LowerLimit=-1*PWMVoltage  OutDataTypeStr=ParamType
  Saturation2 : Saturate  UpperLimit=PWMVoltage  LowerLimit=-1*PWMVoltage  OutDataTypeStr=ParamType
  u_vd : Outport  OutDataTypeStr=ParamType
  u_vq : Outport  Port=2  OutDataTypeStr=ParamType
  wires:
  iq_ref/1 -> MFP_ARDC_1st3/1(r)
  iq/1 -> MFP_ARDC_1st3/2(y)
  Saturation1/1 -> u_vq/1
  MFP_ARDC_1st3/1(u) -> Saturation1/1
  id/1 -> MFP_ARDC_1st2/2(y)
  id_ref/1 -> MFP_ARDC_1st2/1(r)
  MFP_ARDC_1st2/1(u) -> Saturation2/1
  Saturation2/1 -> u_vd/1
  k1_iqd/biq/1 -> MFP_ARDC_1st2/4(k1_iqd/biq), MFP_ARDC_1st3/4(k1_iqd/biq)
  beta_iqd(1)/1 -> MFP_ARDC_1st2/5(beta_iqd(1)), MFP_ARDC_1st3/5(beta_iqd(1))
  beta_iqd(2)/1 -> MFP_ARDC_1st3/6(beta_iqd(2)), MFP_ARDC_1st2/6(beta_iqd(2))
  gam_iqd(1)/1 -> MFP_ARDC_1st2/7(gam_iqd(1)), MFP_ARDC_1st3/7(gam_iqd(1))
  gam_iqd(2)/1 -> MFP_ARDC_1st2/8(gam_iqd(2)), MFP_ARDC_1st3/8(gam_iqd(2))
  alpha_iqd(2)/1 -> MFP_ARDC_1st2/9(alpha_iqd(2)), MFP_ARDC_1st3/9(alpha_iqd(2))
  alpha_iqd(1)/1 -> MFP_ARDC_1st2/10(alpha_iqd(1)), MFP_ARDC_1st3/10(alpha_iqd(1))
  ulim_vd/1 -> MFP_ARDC_1st2/3(ulim)
  ulim_vq/1 -> MFP_ARDC_1st3/3(ulim)

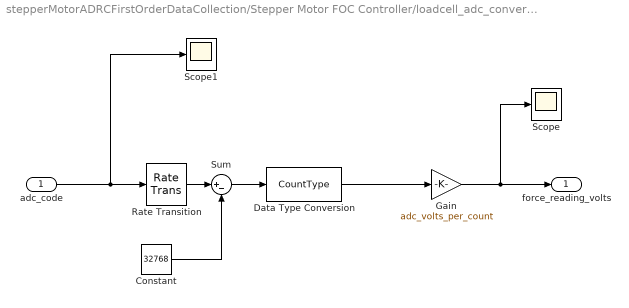
== system stepperMotorADRCFirstOrderDataCollection/Stepper Motor FOC Controller/loadcell_adc_converter ==
  adc_code : Inport  OutMin=[0]  OutDataTypeStr=uint16
  Constant : Constant  Value=32768  OutDataTypeStr=uint16
  Data Type Conversion : DataTypeConversion  OutDataTypeStr=CountType  RndMeth=Floor
  Gain : Gain  Gain=adc_volts_per_count  ParamDataTypeStr=fixdt(0,32,38)  OutDataTypeStr=ParamType  RndMeth=Nearest  SaturateOnIntegerOverflow=on
  Rate Transition : RateTransition  OutPortSampleTime=2e-5
  Scope : Scope
      settings: ActiveDisplayYMinimum=-1  ActiveDisplayYMaximum=1  DataLoggingVariableName=ScopeData3
  Scope1 : Scope
      settings: ActiveDisplayYMinimum=32767.998727508824  ActiveDisplayYMaximum=32768.000120091434  DataLoggingVariableName=ScopeData4
  Sum : Sum  Inputs=|+-  OutDataTypeStr=uint16
  force_reading_volts : Outport  OutDataTypeStr=ParamType
  wires:
  Gain/1 -> Scope/1, force_reading_volts/1
  adc_code/1 -> Scope1/1, Rate Transition/1
  Data Type Conversion/1 -> Gain/1
  Rate Transition/1 -> Sum/1
  Sum/1 -> Data Type Conversion/1
  Constant/1 -> Sum/2

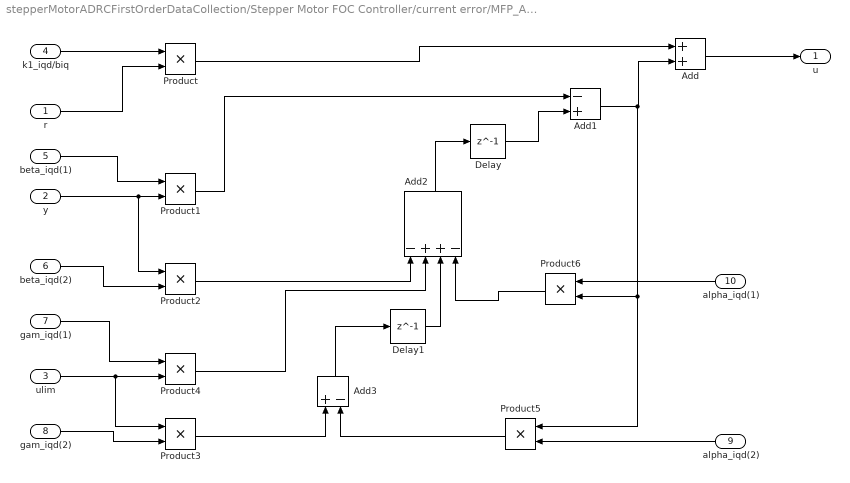
== system stepperMotorADRCFirstOrderDataCollection/Stepper Motor FOC Controller/current error/MFP_ARDC_1st2 ==
  r : Inport
  y : Inport  Port=2
  ulim : Inport  Port=3
  k1_iqd/biq : Inport  Port=4
  beta_iqd(1) : Inport  Port=5
  beta_iqd(2) : Inport  Port=6
  gam_iqd(1) : Inport  Port=7
  gam_iqd(2) : Inport  Port=8
  alpha_iqd(2) : Inport  Port=9
  alpha_iqd(1) : Inport  Port=10
  Add : Sum  SaturateOnIntegerOverflow=on  OutDataTypeStr=Inherit: Same as first input
  Add1 : Sum  Inputs=-+  SaturateOnIntegerOverflow=on  OutDataTypeStr=Inherit: Same as first input
  Add2 : Sum  Inputs=-++-
  Add3 : Sum  Inputs=+-  SaturateOnIntegerOverflow=on  OutDataTypeStr=Inherit: Same as first input
  Delay : Delay  DelayLength=1  InitialCondition=0  SampleTime=2e-5
  Delay1 : Delay  DelayLength=1  InitialCondition=0  SampleTime=2e-5
  Product{,1..6} (7 alike) : Product  SaturateOnIntegerOverflow=on  OutDataTypeStr=Inherit: Same as first input
  u : Outport
  wires:
  Add/1 -> u/1
  Add3/1 -> Delay1/1
  Product4/1 -> Add2/2
  Product6/1 -> Add2/4
  Add1/1 -> Product5/1, Product6/2, Add/2
  Add2/1 -> Delay/1
  r/1 -> Product/2
  Delay1/1 -> Add2/3
  Product3/1 -> Add3/1
  ulim/1 -> Product3/1, Product4/2
  Product2/1 -> Add2/1
  Product5/1 -> Add3/2
  Delay/1 -> Add1/2
  Product1/1 -> Add1/1
  y/1 -> Product2/1, Product1/2
  k1_iqd/biq/1 -> Product/1
  Product/1 -> Add/1
  beta_iqd(1)/1 -> Product1/1
  beta_iqd(2)/1 -> Product2/2
  gam_iqd(1)/1 -> Product4/1
  gam_iqd(2)/1 -> Product3/2
  alpha_iqd(2)/1 -> Product5/2
  alpha_iqd(1)/1 -> Product6/1

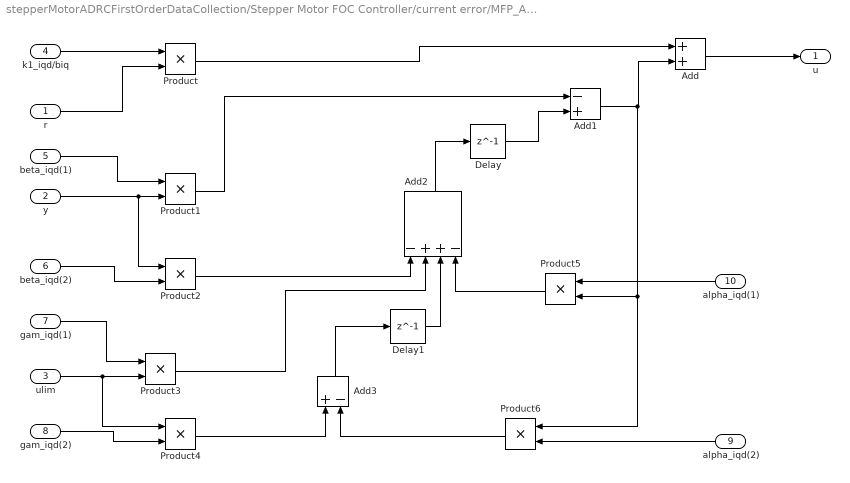
== system stepperMotorADRCFirstOrderDataCollection/Stepper Motor FOC Controller/current error/MFP_ARDC_1st3 ==
  r : Inport
  y : Inport  Port=2
  ulim : Inport  Port=3
  k1_iqd/biq : Inport  Port=4
  beta_iqd(1) : Inport  Port=5
  beta_iqd(2) : Inport  Port=6
  gam_iqd(1) : Inport  Port=7
  gam_iqd(2) : Inport  Port=8
  alpha_iqd(2) : Inport  Port=9
  alpha_iqd(1) : Inport  Port=10
  Add : Sum  SaturateOnIntegerOverflow=on  OutDataTypeStr=Inherit: Same as first input
  Add1 : Sum  Inputs=-+  SaturateOnIntegerOverflow=on  OutDataTypeStr=Inherit: Same as first input
  Add2 : Sum  Inputs=-++-  OutDataTypeStr=CurrLoopType  SaturateOnIntegerOverflow=on
  Add3 : Sum  Inputs=+-  SaturateOnIntegerOverflow=on  OutDataTypeStr=Inherit: Same as first input
  Delay : Delay  DelayLength=1  InitialCondition=0  SampleTime=2e-5
  Delay1 : Delay  DelayLength=1  InitialCondition=0  SampleTime=2e-5
  Product{,1..6} (7 alike) : Product  SaturateOnIntegerOverflow=on  OutDataTypeStr=Inherit: Same as first input
  u : Outport
  wires:
  Add/1 -> u/1
  Add3/1 -> Delay1/1
  Product3/1 -> Add2/2
  Product5/1 -> Add2/4
  Add1/1 -> Product6/1, Product5/2, Add/2
  Add2/1 -> Delay/1
  r/1 -> Product/2
  Delay1/1 -> Add2/3
  Product4/1 -> Add3/1
  ulim/1 -> Product4/1, Product3/2
  Product2/1 -> Add2/1
  Product6/1 -> Add3/2
  Delay/1 -> Add1/2
  Product1/1 -> Add1/1
  y/1 -> Product2/1, Product1/2
  k1_iqd/biq/1 -> Product/1
  Product/1 -> Add/1
  beta_iqd(1)/1 -> Product1/1
  beta_iqd(2)/1 -> Product2/2
  gam_iqd(1)/1 -> Product3/1
  gam_iqd(2)/1 -> Product4/2
  alpha_iqd(2)/1 -> Product6/2
  alpha_iqd(1)/1 -> Product5/1
